simulink model "mat_model_2_telesa"  (R2025b)
settings: Solver=ode45  StartTime=0.0  StopTime=1800  MaxStep=1  RelTol=1e-3
values from neighbouring files (symbols this model uses):
  A = 7e-4    (= 0.0007)    [matlab_2_telesa.m]
  A_int = 12e-4-A    (= 0.0005)    [matlab_2_telesa.m]
  alfa = 0.01    [matlab_2_telesa.m]
  alfa2 = 0.0075    [matlab_2_telesa.m]
  c_p = 500    [matlab_2_telesa.m]
  epsilon = 0.5    [matlab_2_telesa.m]
  m = 0.004    [matlab_2_telesa.m]
  sigma = 5.670374e-8    (= 5.670374e-08)    [matlab_2_telesa.m]
  T_ok = 23 + 273.15    (= 296.15)    [matlab_2_telesa.m]
  T_poc = 23 + 273.15    (= 296.15)    [matlab_2_telesa.m]
  U = 10    [matlab_2_telesa.m]
settings Model: Creator=marob  LastModifiedBy=lukas
settings OptimizationCC: BlockReduction=off  DefaultParameterBehavior=Inlined  BufferReuse=off

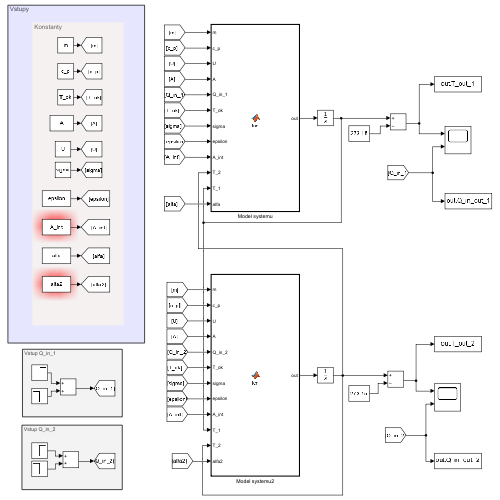
[thumbnail: Simulink's stored preview of the top-level diagram]
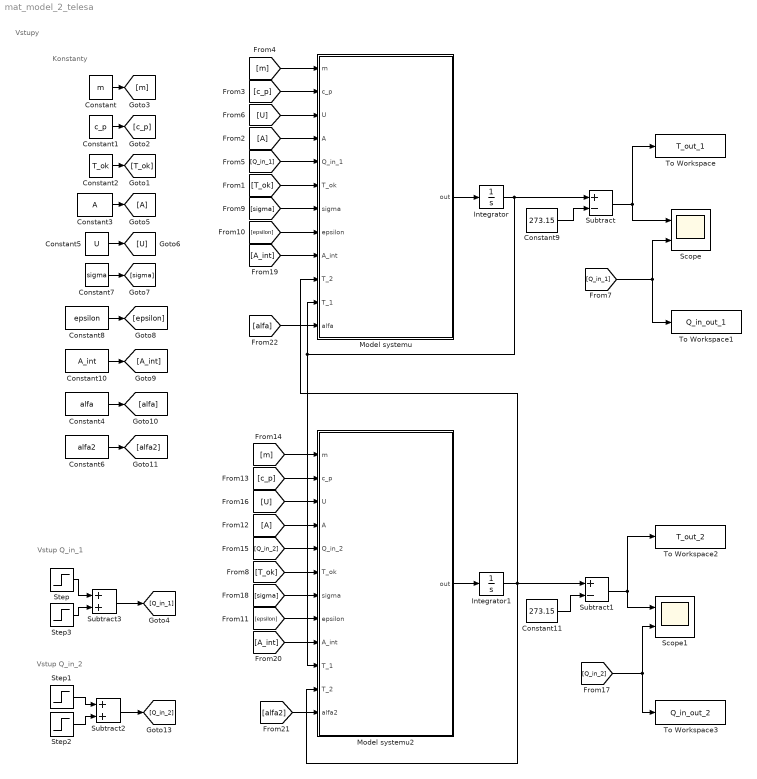
== system mat_model_2_telesa ==
  note: Vstup Q_in_1
  note: Vstupy
  note: Konstanty
  note: Vstup Q_in_2
  Constant : Constant  Value=m
  Constant1 : Constant  Value=c_p
  Constant10 : Constant  Value=A_int
  Constant11 : Constant  Value=273.15
  Constant2 : Constant  Value=T_ok
  Constant3 : Constant  Value=A
  Constant4 : Constant  Value=alfa
  Constant5 : Constant  Value=U
  Constant6 : Constant  Value=alfa2
  Constant7 : Constant  Value=sigma
  Constant8 : Constant  Value=epsilon
  Constant9 : Constant  Value=273.15
  From12 : From
  From2 : From
  Goto5 : Goto
  Integrator : Integrator  InitialCondition=T_poc
  Integrator1 : Integrator  InitialCondition=T_poc
  Model systemu : MATLAB Function  TreatAsAtomicUnit=on
  Model systemu2 : MATLAB Function  TreatAsAtomicUnit=on
  Scope : Scope  NumInputPorts=2
      settings: ActiveDisplayYMinimum=-5.7807366194750989  ActiveDisplayYMaximum=52.0266295752759
  Scope1 : Scope  NumInputPorts=2
      settings: ActiveDisplayYMinimum=-5.7807366194750989  ActiveDisplayYMaximum=52.0266295752759
  Step : Step  After=50  SampleTime=0
  Step1 : Step  Time=900  After=40  SampleTime=0
  Step2 : Step  Time=1500  After=-40  SampleTime=0
  Step3 : Step  Time=900  After=-50  SampleTime=0
  Subtract : Sum  Inputs=+-
  Subtract1 : Sum  Inputs=+-
  Subtract2 : Sum
  Subtract3 : Sum
  To Workspace : ToWorkspace  VariableName=T_out_1  SaveFormat=Timeseries  SampleTime=-1
  To Workspace1 : ToWorkspace  VariableName=Q_in_out_1  SaveFormat=Timeseries  SampleTime=-1
  To Workspace2 : ToWorkspace  VariableName=T_out_2  SaveFormat=Timeseries  SampleTime=-1
  To Workspace3 : ToWorkspace  VariableName=Q_in_out_2  SaveFormat=Timeseries  SampleTime=-1
  wires:
  Model systemu/1(out) -> Integrator/1
  Constant2/1 -> [T_ok]
  Constant/1 -> [m]
  Constant1/1 -> [c_p]
  [c_p] -> Model systemu/2(c_p)
  [m] -> Model systemu/1(m)
  Integrator/1 -> Subtract/1, Model systemu/11(T_1), Model systemu2/10(T_1)
  [Q_in_1] -> Model systemu/5(Q_in_1)
  [T_ok] -> Model systemu/6(T_ok)
  Constant3/1 -> Goto5/1
  Constant5/1 -> [U]
  [U] -> Model systemu/3(U)
  From2/1 -> Model systemu/4(A)
  [Q_in_1] -> To Workspace1/1, Scope/2
  Subtract/1 -> To Workspace/1, Scope/1
  Constant9/1 -> Subtract/2
  Constant7/1 -> [sigma]
  [sigma] -> Model systemu/7(sigma)
  Constant8/1 -> [epsilon]
  [epsilon] -> Model systemu/8(epsilon)
  Constant10/1 -> [A_int]
  Subtract1/1 -> Scope1/1, To Workspace2/1
  [sigma] -> Model systemu2/7(sigma)
  [Q_in_2] -> Model systemu2/5(Q_in_2)
  From12/1 -> Model systemu2/4(A)
  [Q_in_2] -> To Workspace3/1, Scope1/2
  [U] -> Model systemu2/3(U)
  Constant11/1 -> Subtract1/2
  [m] -> Model systemu2/1(m)
  Integrator1/1 -> Model systemu2/11(T_2), Subtract1/1, Model systemu/10(T_2)
  [epsilon] -> Model systemu2/8(epsilon)
  [c_p] -> Model systemu2/2(c_p)
  [T_ok] -> Model systemu2/6(T_ok)
  Model systemu2/1(out) -> Integrator1/1
  [A_int] -> Model systemu/9(A_int)
  [A_int] -> Model systemu2/9(A_int)
  Step1/1 -> Subtract2/1
  Step2/1 -> Subtract2/2
  Subtract2/1 -> [Q_in_2]
  Subtract3/1 -> [Q_in_1]
  Step/1 -> Subtract3/1
  Step3/1 -> Subtract3/2
  Constant4/1 -> [alfa]
  [alfa2] -> Model systemu2/12(alfa2)
  [alfa] -> Model systemu/12(alfa)
  Constant6/1 -> [alfa2]

== matlab function mat_model_2_telesa/Model systemu2 ==
  data: m input; out output; c_p input; U input; A input; Q_in_2 input; T_ok input; sigma input; epsilon input; A_int input; T_1 input; T_2 input; alfa2 input
function out = fcn(m, c_p, U, A, Q_in_2, T_ok, sigma, epsilon, A_int, T_1, T_2, alfa2)


out = (1/(m*c_p)) * (alfa2*Q_in_2 - U*A*(T_2-T_ok) - sigma*epsilon*A*( (T_2^4) - (T_ok^4) ) + A_int * U * (T_1 - T_2) + sigma*epsilon*A_int*(T_1^4 - T_2^4) );

== matlab function mat_model_2_telesa/Model systemu ==
  data: m input; out output; c_p input; U input; A input; Q_in_1 input; T_ok input; sigma input; epsilon input; A_int input; T_2 input; T_1 input; alfa input
function out = fcn(m, c_p, U, A, Q_in_1, T_ok, sigma, epsilon, A_int, T_2, T_1, alfa)

out = (1/(m*c_p)) * (alfa*Q_in_1 - U*A*(T_1-T_ok) - sigma*epsilon*A*( (T_1^4) - (T_ok^4) ) - A_int * U * (T_1 - T_2) - sigma*epsilon*A_int*(T_1^4 - T_2^4) );
